simulink model "FSI01_02"  (R2024b)
settings: Solver=VariableStepAuto  StartTime=0.0  StopTime=5  MaxStep=1e-3  RelTol=1e-3
values from neighbouring files (symbols this model uses):
  a = out.ScopeData2.signals(1).values    [FSI01WS.m]
  v0 = 25    [FSI01WS.m]    (also in FSI08WS.m = 0; FSI09WS.m = 0)
settings Model: Creator=fmiro  LastModifiedBy=fmiro

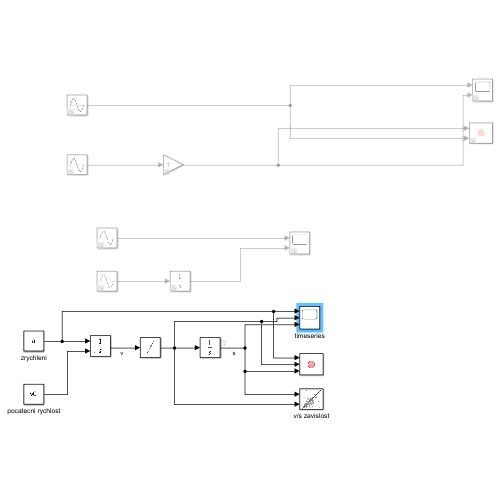
[thumbnail: Simulink's stored preview of the top-level diagram]
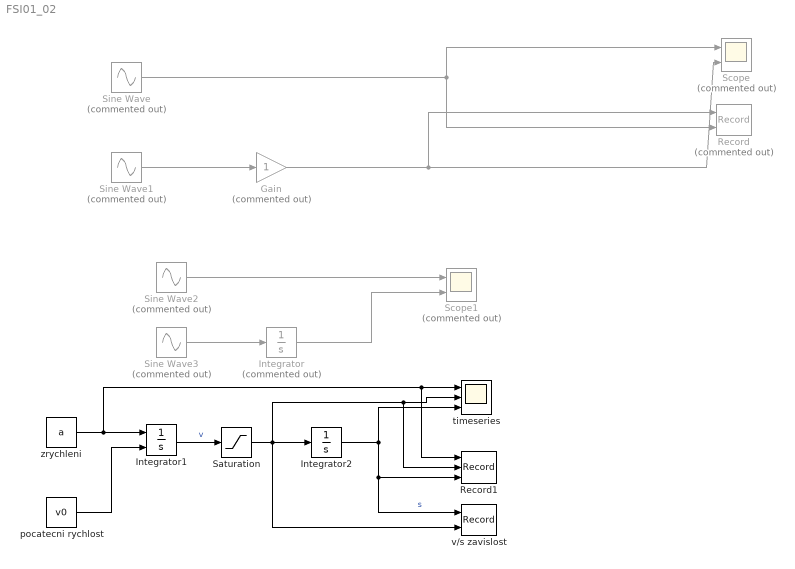
== system FSI01_02 ==
  Gain : Gain  Commented=on
  Integrator : Integrator  Commented=on
  Integrator1 : Integrator  InitialConditionSource=external
  Integrator2 : Integrator
  Record : Record  Commented=on  FileSettingsInternal="{\"entries\":[{\"content\":{\"excelSettings\":{\"content\":{},\"type\":\"Streamout.ExcelSettings\"}},\"type\":\"Streamout.FileSettingStorage\",\"uuid\":\"\"}],\"packageUris\":[\"http:\\/\\/schema.mathworks.com\\/mf0\\/streamout_blocks\\/R2020a\"],\"version\":\"1.0\"}"  SignalsInternal="{\"entries\":[{\"content\":{},\"type\":\"RecordBlkView.InputSignals\",\"uuid\":\"\"}],\"packageUris\":[\"http:\\/\\/schema.mathworks.com\\/mf0\\/streamout_blocks\\/R2020a\"],\"version\":\"1.0\"}"  VisualizationBindings="{\"sparklinesplugin\":{\"info\":[{\"bindingParametersList\":[],\"subplotID\":1}]}}"
  Record1 : Record  FileSettingsInternal="{\"entries\":[{\"content\":{\"excelSettings\":{\"content\":{},\"type\":\"Streamout.ExcelSettings\"}},\"type\":\"Streamout.FileSettingStorage\",\"uuid\":\"\"}],\"packageUris\":[\"http:\\/\\/schema.mathworks.com\\/mf0\\/streamout_blocks\\/R2020a\"],\"version\":\"1.0\"}"  SignalsInternal="{\"entries\":[{\"content\":{\"signals\":[{\"content\":{\"blockPath\":[],\"dimensions\":[1],\"domain\":\"\",\"lineColor\":\"#4dbeee\",\"lineWidth\":2,\"plots\":[ 1 ],\"port\":2,\"sid\":[\"\"],\"signalID\":1,\"signalName\":\"Saturation\"},\"type\":\"RecordBlkView.Signal\",\"uuid\":\"\"},{\"content\":{\"blockPath\":[],\"dimensions\":[1],\"domain\":\"\",\"lineColor\":\"#64d413\",\"lineWidth\":2,\"plots\":[ 1 ],\"port\":3,\"sid\":[\"\"],\"signalID\":2,\"signalName\":\"s\"},\"type\":\"RecordBlkView.Signal\",\"uuid\":\"\"},{\"content\":{\"blockPath\":[],\"dimensions\":[1],\"domain\":\"\",\"lineColor\":\"#77ac30\",\"lineWidth\":2,\"plots\":[ 1 ],\"port\":1,\"sid\":[\"\"],\"signalID\":3,\"signalName\":\"zrychleni\"},\"type\":\"RecordBlkView.Signal\",\"uuid\":\"\"}]},\"type\":\"RecordBlkView.InputSignals\",\"uuid\":\"\"}],\"packageUris\":[\"http:\\/\\/schema.mathworks.com\\/mf0\\/streamout_blocks\\/R2020a\"],\"version\":\"1.0\"}"  VisualizationBindings="{\"sparklinesplugin\":{\"info\":[{\"bindingParametersList\":[],\"subplotID\":1}]}}"
  Saturation : Saturate  UpperLimit=inf  LowerLimit=0
  Scope : Scope  Commented=on  NumInputPorts=2
  Scope1 : Scope  Commented=on  NumInputPorts=2
  Sine Wave : Sin  Commented=on  SampleTime=0
  Sine Wave1 : Sin  Commented=on  Phase=pi  SampleTime=0
  Sine Wave2 : Sin  Commented=on  SampleTime=0
  Sine Wave3 : Sin  Commented=on  SampleTime=0
  pocatecni rychlost : Constant  Value=v0
  timeseries : Scope  NumInputPorts=3
  v/s zavislost : Record  FileSettingsInternal="{\"entries\":[{\"content\":{\"excelSettings\":{\"content\":{},\"type\":\"Streamout.ExcelSettings\"}},\"type\":\"Streamout.FileSettingStorage\",\"uuid\":\"\"}],\"packageUris\":[\"http:\\/\\/schema.mathworks.com\\/mf0\\/streamout_blocks\\/R2020a\"],\"version\":\"1.0\"}"  Layout=[1 1]  SignalsInternal="{\"entries\":[{\"content\":{\"signals\":[{\"content\":{\"blockPath\":[],\"dimensions\":[1],\"domain\":\"\",\"lineColor\":\"#139fff\",\"lineWidth\":2,\"port\":1,\"sid\":[\"\"],\"signalID\":1,\"signalName\":\"s\"},\"type\":\"RecordBlkView.Signal\",\"uuid\":\"\"},{\"content\":{\"blockPath\":[],\"dimensions\":[1],\"domain\":\"\",\"lineColor\":\"#139fff\",\"plots\":[ 1 ],\"port\":2,\"sid\":[\"\"],\"signalID\":2,\"signalName\":\"Saturation\"},\"type\":\"RecordBlkView.Signal\",\"uuid\":\"\"}]},\"type\":\"RecordBlkView.InputSignals\",\"uuid\":\"\"}],\"packageUris\":[\"http:\\/\\/schema.mathworks.com\\/mf0\\/streamout_blocks\\/R2020a\"],\"version\":\"1.0\"}"  VisualizationBindings="{\"xyplotplugin\":{\"info\":[{\"series\":[{\"bindingParametersList\":[{\"parameter\":\"Y-Axis\",\"signalID\":2,\"signalName\":\"Saturation\"}],\"seriesID\":0}],\"subplotID\":1}]}}"  CompatibilityTag=XY
  zrychleni : Constant  Value=a
  wires:
  Sine Wave/1 -> Scope/1, Record/2
  Sine Wave1/1 -> Gain/1
  Gain/1 -> Record/1, Scope/2
  Sine Wave3/1 -> Integrator/1
  Integrator/1 -> Scope1/2
  Sine Wave2/1 -> Scope1/1
  zrychleni/1 -> Record1/1, timeseries/1, Integrator1/1
  pocatecni rychlost/1 -> Integrator1/2
  Integrator1/1 -> Saturation/1  "v"
  Integrator2/1 -> Record1/3, v/s zavislost/1, timeseries/3  "s"
  Saturation/1 -> Integrator2/1, Record1/2, timeseries/2, v/s zavislost/2
